simulink model "alvik_battery_example"  (R2026b)
settings: Solver=FixedStepDiscrete  StopTime=Inf  FixedStep=0.02  EnableMultiTasking=on
values from neighbouring files (symbols this model uses):
  s = coder.ceval('MW_Alvik_Status')    [AlvikRobot.m]
libraries: AlvikBlocks x1
settings Model: SILPILModeSetting=veronly  Creator=arkad  LastModifiedBy=arkad
settings SolverCC: AutoInsertRateTranBlk=on
settings OptimizationCC: DifferentSizesBufferReuse=on  EfficientTunableParamExpr=on  EnhancedBackFolding=on  MaxStackSize=64  OptimizationCustomize=off  OptimizeBlockOrder=speed  PassReuseOutputArgsAs=Individual arguments  RemoveInternalMemoryZeroInit=on  RemoveRootLevelIOMemoryZeroInit=on
settings DebuggingCC: ParameterTunabilityLossMsg=error
settings HardwareCC: ProdHWDeviceType=ARM Compatible->ARM Cortex  ProdLargestAtomicFloat=Double  ProdLargestAtomicInteger=Long
settings SFSimCC: MATLABDynamicMemAlloc=off
settings RTWCC: BuildConfiguration=Faster Runs  Description=Embedded Coder  HardwareBoard=Arduino Nano ESP32  SystemTargetFile=ert.tlc  TLCOptions="-aInlineSetEventsForThisBaseRateFcn=TLC_FALSE -aSuppressMultiTaskScheduler=TLC_FALSE  -aRateBasedStepFcn=0"  TemplateMakefile=ert_default_tmf  Toolchain=ESP32
settings CodeAppCC: ForceParamTrailComments=on  IgnoreCustomStorageClasses=off  InsertBlockDesc=on  OperatorAnnotations=on  SFDataObjDesc=on  SimulinkDataObjDesc=on
settings ERTTargetCC: CombineSignalStateStructs=on  ExtModeAutomaticAllocSize=off  ExtModeIntrfLevel=Level2 - Open  ExtModeMexFile=ext_xcp  ExtModeStaticAlloc=on  SupportContinuousTime=on  SupportVariableSizeSignals=on

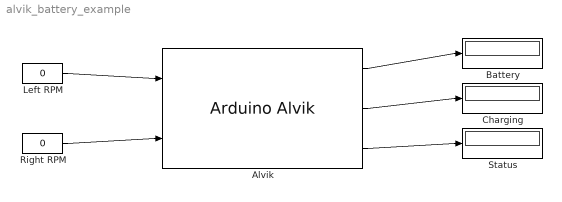
== system alvik_battery_example ==
  Alvik : AlvikBlocks/Arduino Alvik  SampleTime=0.02  BatterySampleTime=1  OutputCharging=on  OutputStatus=on  MotorMode=Wheel speeds (left, right)  WheelUnits=RPM  WheelLimit=Inf  LinearUnits=cm/s  AngularUnits=deg/s  LinearLimit=Inf  AngularLimit=Inf
      settings: SourceProductName=Arduino Alvik
  Battery : Display
  Charging : Display
  Left RPM : Constant  Value=0
  Right RPM : Constant  Value=0
  Status : Display
  wires:
  Left RPM/1 -> Alvik/1
  Right RPM/1 -> Alvik/2
  Alvik/1 -> Battery/1
  Alvik/2 -> Charging/1
  Alvik/3 -> Status/1
